simulink model "suspension"  (R2026a)
settings: Solver=FixedStepAuto  FixedStep=1/1000
values from neighbouring files (symbols this model uses):
  b1 = 87.5    [Automotive_suspension_parameters.m]    (also in parametres_suspension.m)
  b2 = 3755    [Automotive_suspension_parameters.m]    (also in parametres_suspension.m)
  k1 = 20000    [Automotive_suspension_parameters.m]    (also in parametres_suspension.m)
  k2 = 125000    [Automotive_suspension_parameters.m]    (also in parametres_suspension.m)
  m1 = 500    [Automotive_suspension_parameters.m]    (also in parametres_suspension.m)
  m2 = 80    [Automotive_suspension_parameters.m]    (also in parametres_suspension.m)
undefined symbols (not defined in the file or in its folder): F, w
settings Model: Creator=lulu1  LastModifiedBy=lulu1

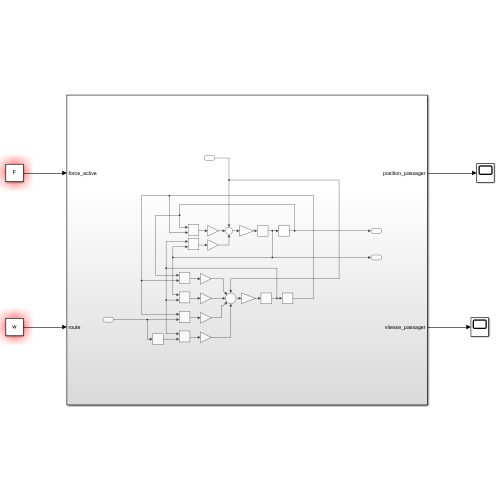
[thumbnail: Simulink's stored preview of the top-level diagram]
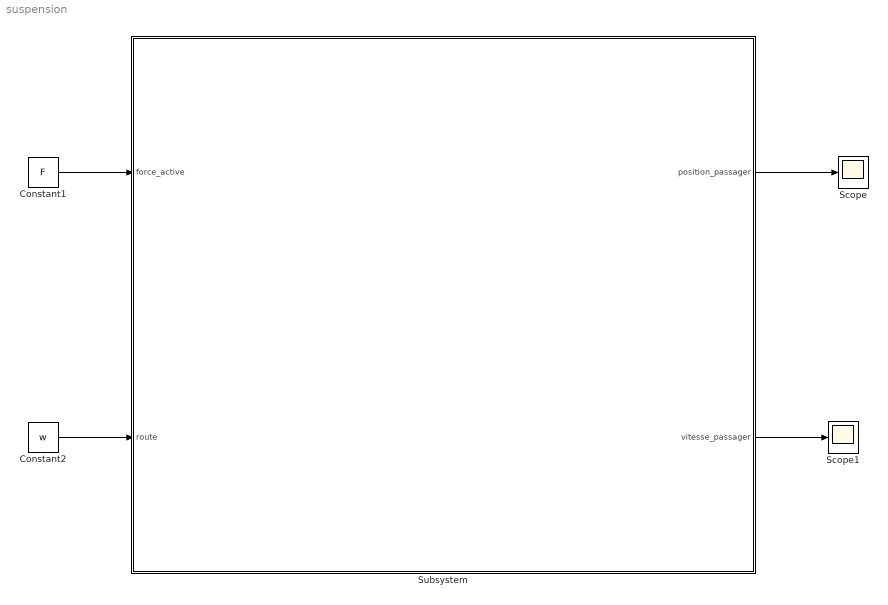
== system suspension ==
  Constant1 : Constant  Value=F
  Constant2 : Constant  Value=w
  Scope : Scope
  Scope1 : Scope
  Subsystem : Subsystem
  wires:
  Constant1/1 -> Subsystem/1(force_active)
  Constant2/1 -> Subsystem/2(route)
  Subsystem/1(position_passager) -> Scope/1
  Subsystem/2(vitesse_passager) -> Scope1/1

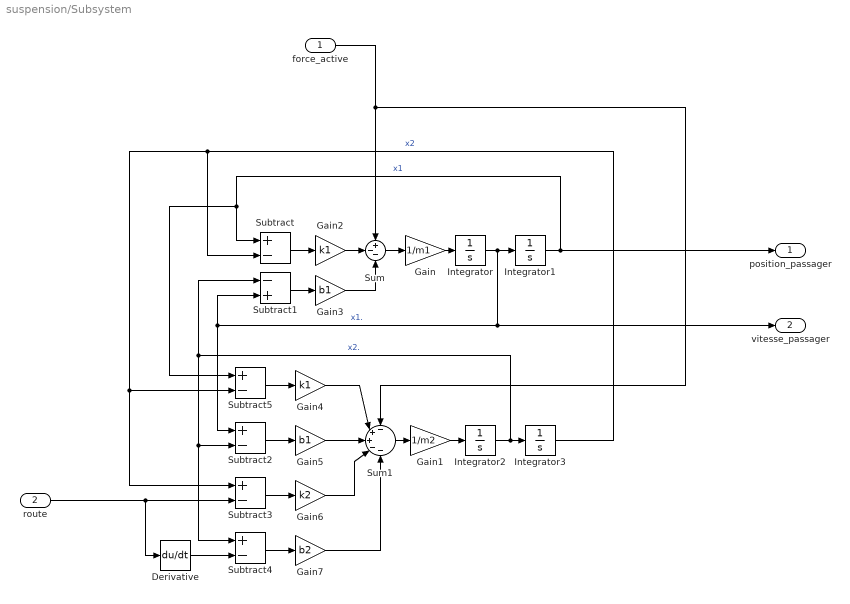
== system suspension/Subsystem ==
  force_active : Inport
  route : Inport  Port=2
  Derivative : Derivative
  Gain : Gain  Gain=1/m1
  Gain1 : Gain  Gain=1/m2
  Gain2 : Gain  Gain=k1
  Gain3 : Gain  Gain=b1
  Gain4 : Gain  Gain=k1
  Gain5 : Gain  Gain=b1
  Gain6 : Gain  Gain=k2
  Gain7 : Gain  Gain=b2
  Integrator{,1..3} (4 alike) : Integrator
  Subtract{,2..5} (5 alike) : Sum  Inputs=+-
  Subtract1 : Sum  Inputs=-+
  Sum : Sum  Inputs=+--
  Sum1 : Sum  Inputs=-++--
  position_passager : Outport
  vitesse_passager : Outport  Port=2
  wires:
  Integrator3/1 -> Subtract/2, Subtract5/2, Subtract3/1  "x2"
  Gain5/1 -> Sum1/3
  Subtract2/1 -> Gain5/1
  Integrator1/1 -> position_passager/1, Subtract/1, Subtract5/1  "x1"
  Integrator2/1 -> Integrator3/1, Subtract4/1, Subtract2/2, Subtract1/1  "x2."
  Integrator/1 -> Integrator1/1, Subtract2/1, Subtract1/2, vitesse_passager/1  "x1."
  Derivative/1 -> Subtract4/2
  Sum/1 -> Gain/1
  Gain1/1 -> Integrator2/1
  Gain7/1 -> Sum1/5
  Gain6/1 -> Sum1/4
  Subtract4/1 -> Gain7/1
  Gain4/1 -> Sum1/2
  route/1 -> Subtract3/2, Derivative/1
  Subtract5/1 -> Gain4/1
  Subtract3/1 -> Gain6/1
  Subtract1/1 -> Gain3/1
  Gain/1 -> Integrator/1
  Gain3/1 -> Sum/3
  Gain2/1 -> Sum/2
  Subtract/1 -> Gain2/1
  force_active/1 -> Sum1/1, Sum/1
  Sum1/1 -> Gain1/1
